simulink model "Greenhouse_Temp_Control"  (R2023b)
settings: Solver=VariableStepAuto  StartTime=0.0  StopTime=24.0  RelTol=1e-3
undefined symbols (not defined in the file or in its folder): Kd, Ki, Kp
libraries: SignalEditorBlockLib x2, eeGeneralControl x1, spspowerguiLib x1
settings Model: Creator=danbr  LastModifiedBy=danbr

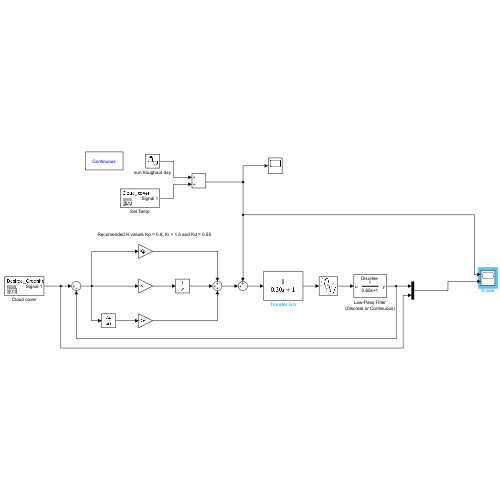
[thumbnail: Simulink's stored preview of the top-level diagram]
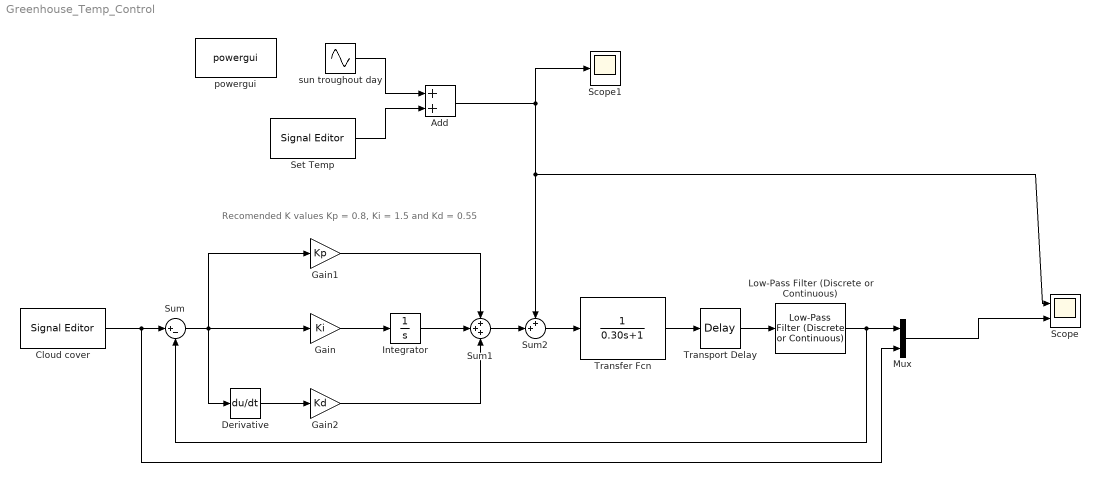
== system Greenhouse_Temp_Control ==
  note: Recomended K values Kp = 0.8, Ki = 1.5 and Kd = 0.55
  Add : Sum
  Cloud cover : SignalEditorBlockLib/Signal Editor  FileName=C:\Users\danbr\OneDrive - Cardiff Metropolitan University\ADV control systems\Greenhouse_Temp_Desired.mat  ActiveScenario=Desired_Greenhouse_Temp  ActiveSignal=Signal 1  IsBus=off  OutputBusObjectStr=Bus: BusObject  SampleTime=0  Interpolate=off  ZeroCross=off  OutputAfterFinalValue=Setting to zero  Unit=inherit  PreserveSignalName=on  ApplySigPropsToAllScenarios=off  ApplySigPropsToAllSignals=off
  Derivative : Derivative
  Gain : Gain  Gain=Ki
  Gain1 : Gain  Gain=Kp
  Gain2 : Gain  Gain=Kd
  Integrator : Integrator
  Low-Pass Filter (Discrete or Continuous) : eeGeneralControl/Low-Pass Filter (Discrete or Continuous)  K=1  T=0.65  B=inf  A=-inf  init_option=Inherited from block input  x0=0  Ts=-1
  Mux : Mux  Inputs=2
  Scope : Scope  NumInputPorts=2
  Scope1 : Scope
  Set Temp : SignalEditorBlockLib/Signal Editor  FileName=C:\Users\danbr\OneDrive - Cardiff Metropolitan University\ADV control systems\Cloud cover.mat  ActiveScenario=Cloud_cover  ActiveSignal=Signal 1  IsBus=off  OutputBusObjectStr=Bus: BusObject  SampleTime=0  Interpolate=off  ZeroCross=off  OutputAfterFinalValue=Setting to zero  Unit=inherit  PreserveSignalName=on  ApplySigPropsToAllScenarios=off  ApplySigPropsToAllSignals=off
  Sum : Sum  Inputs=|+-
  Sum1 : Sum  Inputs=+++
  Sum2 : Sum  Inputs=++|
  Transfer Fcn : TransferFcn  Denominator=[0.30 1]
  Transport Delay : TransportDelay  DelayTime=0.15
  powergui : spspowerguiLib/powergui  Priority=1  SimulationMode=Continuous  SampleTime=50e-6  frequency=60  Iterations=50  frequencyindice=60  Pbase=100e6  ErrMax=1e-4  UnitsV=kV  UnitsW=MW  buscounter=0  FunctionMessages=off  echomessages=off  EnableUseOfTLC=off  CurrentSourceSwitches=off  DisableSnubberDevices=off  DisableRonSwitches=off  DisableVfSwitches=off  DisplayEquations=off  AutomaticDiscreteSolvers=off  SolverType=Tustin/Backward Euler (TBE)  Interpol=off  ExternalGateDelay=off  methode=off  Ts=100  x0status=blocks  SPID=on  SwTol=0  HookPort=off  NonlinearTolerance=1e-4  nMaxIteration=100  ContinueOnMaxIteration=off  RestoreLinks=warning  ResistiveCurrentMeasurement=off  Frange=[0:2:500]  Ylog=off  Xlog=on  ShowGrid=off  save=off  variable=ZData  structure=0  ZoomFFT=off  StartTime=0.0  cycles=1  DisplayStyle=1  fundamental=60  FreqAxis=off  MaxFrequency=1000  frequencyindicesteady=1  RmsSteady=1  display=off
  sun troughout day : Sin  Amplitude=10  Bias=12  Frequency=2*pi/24  Phase=3*pi/2  SampleTime=0.1
  wires:
  sun troughout day/1 -> Add/1
  Set Temp/1 -> Add/2
  Cloud cover/1 -> Mux/2, Sum/1
  Gain1/1 -> Sum1/1
  Integrator/1 -> Sum1/2
  Gain/1 -> Integrator/1
  Derivative/1 -> Gain2/1
  Sum/1 -> Derivative/1, Gain1/1, Gain/1
  Add/1 -> Scope/1, Sum2/1, Scope1/1
  Sum2/1 -> Transfer Fcn/1
  Sum1/1 -> Sum2/2
  Mux/1 -> Scope/2
  Transfer Fcn/1 -> Transport Delay/1
  Gain2/1 -> Sum1/3
  Transport Delay/1 -> Low-Pass Filter (Discrete or Continuous)/1
  Low-Pass Filter (Discrete or Continuous)/1 -> Mux/1, Sum/2
